simulink model "FOC_LADRC_G474_bias_isolated_v2"  (R2020b)
settings: Solver=FixedStepDiscrete  StartTime=0.0  StopTime=10  FixedStep=TsBSP  RelTol=1e-3
values from neighbouring files (symbols this model uses):
  BandwidthCurrentPI = 1256.6370614359173    [G474_FOC_LADRC.sldd]
  Flux = 0.0109    [G474_FOC_LADRC.sldd]
  Flux_MODEL = 0.0109    [G474_FOC_LADRC.sldd]
  LADRC_b0 = 8000.0    [G474_FOC_LADRC.sldd]
  LADRC_Omega_c = 150.0    [G474_FOC_LADRC.sldd]
  Ls = 0.000195185    [G474_FOC_LADRC.sldd]
  MaxVoltage = 10.0    [G474_FOC_LADRC.sldd]
  pll_omega = 5000.0    [G474_FOC_LADRC.sldd]
  pll_xi = 10.0    [G474_FOC_LADRC.sldd]
  PolePairs = 5.0    [G474_FOC_LADRC.sldd]
  PolePairs_MODEL = 5.0    [G474_FOC_LADRC.sldd]
  PWMHalfPeriod = 4199.0    [G474_FOC_LADRC.sldd]
  Rs = 0.1763    [G474_FOC_LADRC.sldd]
  TsBSP = 2.5E-5    [G474_FOC_LADRC.sldd]
  TsBSP_MODEL = 2.5E-5    [G474_FOC_LADRC.sldd]
  TsFOC = 0.0001    [G474_FOC_LADRC.sldd]
  TsFOC_MODEL = 0.0001    [G474_FOC_LADRC.sldd]
undefined symbols (not defined in the file or in its folder): DiscIntNeverNeededParam, magnitude, sigbuilder_block
libraries: slpidlib x3, mcbplantlib x1, autolibpmsmexterior x1
PreSaveFcn:
  | cd(fileparts(which(bdroot)));
settings Model: DataDictionary=G474_FOC_LADRC.sldd  PacingRate=1000  Creator=beau_  LastModifiedBy=admin
settings DataIOCC: SaveOutput=off  DSMLogging=off  SaveTime=off  ReturnWorkspaceOutputs=off
settings OptimizationCC: DefaultParameterBehavior=Inlined  EnhancedBackFolding=on  PassReuseOutputArgsAs=Individual arguments  ZeroExternalMemoryAtStartup=off  OptimizeBlockOrder=speed  DifferentSizesBufferReuse=on  OptimizationCustomize=off  EfficientTunableParamExpr=on
settings DebuggingCC: SignalRangeChecking=warning  ParameterPrecisionLossMsg=none  ParameterTunabilityLossMsg=error
settings HardwareCC: ProdBitPerPointer=32  ProdBitPerSizeT=32  ProdBitPerPtrDiffT=32  ProdLargestAtomicInteger=Long  ProdLargestAtomicFloat=Double  ProdWordSize=32  ProdHWDeviceType=ARM Compatible->ARM Cortex-M
settings SFSimCC: SimParseCustomCode=off  MATLABDynamicMemAlloc=off
settings RTWCC: Description=Embedded Coder  SystemTargetFile=ert.tlc  GenCodeOnly=on  TemplateMakefile=ert_default_tmf  RTWUseSimCustomCode=on
settings CodeAppCC: ForceParamTrailComments=on  GenerateComments=off  IgnoreCustomStorageClasses=off  OperatorAnnotations=on  SimulinkDataObjDesc=on  SFDataObjDesc=on  InsertBlockDesc=on
settings ERTTargetCC: TargetLangStandard=C99 (ISO)  CodeReplacementLibrary=ARM Cortex-M  GenerateSampleERTMain=on  SupportAbsoluteTime=off  SupportNonFinite=off  SupportComplex=off  InlinedParameterPlacement=NonHierarchical  ERTCustomFileTemplate=example_file_process.tlc  IndentSize=4

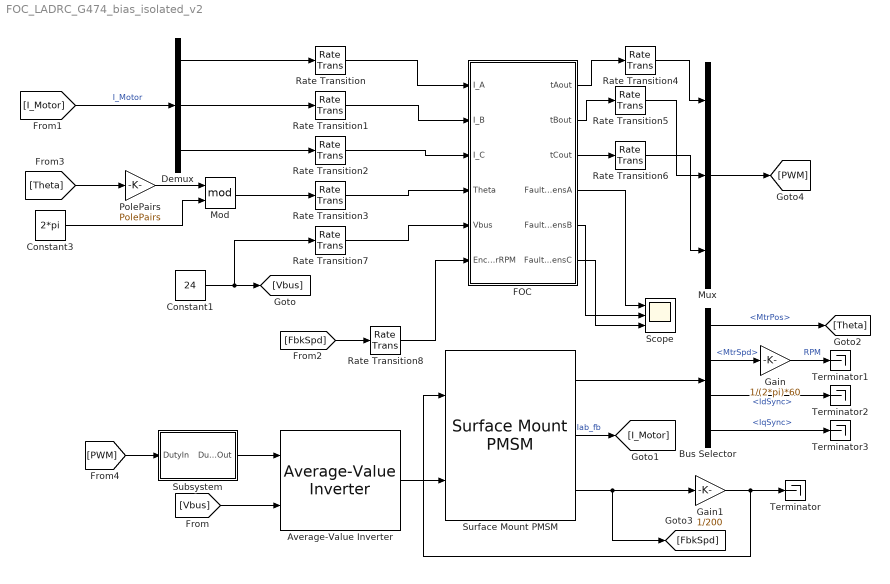
== system FOC_LADRC_G474_bias_isolated_v2 ==
  Average-Value Inverter : mcbplantlib/Average-Value Inverter
  Bus Selector : BusSelector  OutputSignals=MtrPos,MtrSpd,IdSync,IqSync
  Constant1 : Constant  Value=24  SampleTime=TsBSP
  Constant3 : Constant  Value=2*pi  SampleTime=TsBSP
  Demux : Demux  Outputs=3
  FOC : Subsystem  SystemSampleTime=TsFOC
  Gain : Gain  Gain=1/(2*pi)*60
  Gain1 : Gain  Gain=1/200
  Mod : Math  Operator=mod  SaturateOnIntegerOverflow=on
  Mux : Mux  Inputs=3
  PolePairs : Gain  Gain=PolePairs
  Rate Transition{,1..3,7..8} (6 alike) : RateTransition
  Rate Transition4 : RateTransition  OutPortSampleTime=TsBSP
  Rate Transition5 : RateTransition  OutPortSampleTime=TsBSP
  Rate Transition6 : RateTransition  OutPortSampleTime=TsBSP
  Scope : Scope  NumInputPorts=3
  Subsystem : Subsystem
  Surface Mount PMSM : autolibpmsmexterior/Surface Mount PMSM  port_config=Torque  sim_type=Discrete  Ts=TsBSP_MODEL  P=PolePairs_MODEL  Rs=Rs_MODEL  Ldq_=Ls_MODEL  KConstText=Permanent flux linkage constant (lambda_pm):  lambda_pm=Flux_MODEL  Ke=0.0419  Kt=0.061  mechanical=[2.8e-4, 1e-5, 0]  idq0=[0 0]  theta_init=0  omega_init=5  KConst=Flux_MODEL  lambda_pm_calc=Flux_MODEL  RefBlkName='autolibpmsmexterior/Surface Mount PMSM'  aMode=5  Ldq="[0.0017      0.0017]"
      settings: SourceProductBaseCode=PW,MT,UV,VE,VP
  Terminator{,1..3} (4 alike) : Terminator
  wires:
  Average-Value Inverter/1 -> Surface Mount PMSM/2
  Rate Transition4/1 -> Mux/1
  Surface Mount PMSM/2 -> [I_Motor]  "Iab_fb"
  Rate Transition7/1 -> FOC/5(Vbus)
  Surface Mount PMSM/3 -> [FbkSpd], Gain1/1
  Bus Selector/4 -> Terminator3/1  "<IqSync>"
  Bus Selector/3 -> Terminator2/1  "<IdSync>"
  [Vbus] -> Average-Value Inverter/2
  Mux/1 -> [PWM]
  Rate Transition2/1 -> FOC/3(I_C)
  Mod/1 -> Rate Transition3/1
  PolePairs/1 -> Mod/1
  Subsystem/1(DutyOut) -> Average-Value Inverter/1
  Constant1/1 -> Rate Transition7/1, [Vbus]
  Rate Transition3/1 -> FOC/4(Theta)
  Demux/3 -> Rate Transition2/1
  Rate Transition/1 -> FOC/1(I_A)
  Demux/1 -> Rate Transition/1
  Gain1/1 -> Surface Mount PMSM/1, Terminator/1
  Rate Transition5/1 -> Mux/2
  Surface Mount PMSM/1 -> Bus Selector/1
  Rate Transition6/1 -> Mux/3
  Bus Selector/1 -> [Theta]  "<MtrPos>"
  FOC/2(tBout) -> Rate Transition5/1
  [Theta] -> PolePairs/1
  FOC/3(tCout) -> Rate Transition6/1
  FOC/1(tAout) -> Rate Transition4/1
  Demux/2 -> Rate Transition1/1
  Bus Selector/2 -> Gain/1  "<MtrSpd>"
  Constant3/1 -> Mod/2
  Rate Transition1/1 -> FOC/2(I_B)
  [PWM] -> Subsystem/1(DutyIn)
  [I_Motor] -> Demux/1  "I_Motor"
  Gain/1 -> Terminator1/1  "RPM"
  [FbkSpd] -> Rate Transition8/1
  Rate Transition8/1 -> FOC/6(EncoderRPM)
  FOC/4(Fault_ISensA) -> Scope/1
  FOC/5(Fault_ISensB) -> Scope/2
  FOC/6(Fault_ISensC) -> Scope/3

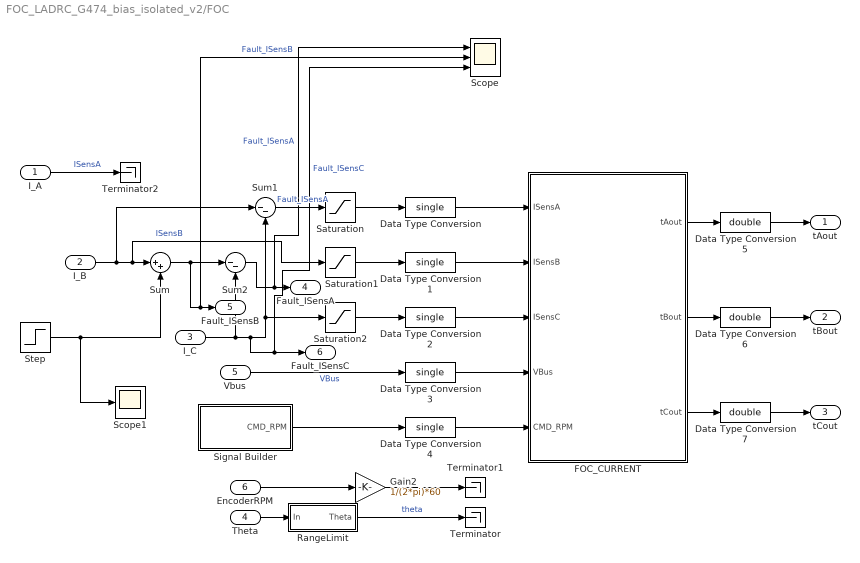
== system FOC_LADRC_G474_bias_isolated_v2/FOC ==
  I_A : Inport
  I_B : Inport  Port=2
  I_C : Inport  Port=3
  Theta : Inport  Port=4
  Vbus : Inport  Port=5
  EncoderRPM : Inport  Port=6
  Data Type Conversion{,1..4} (5 alike) : DataTypeConversion  OutDataTypeStr=single
  Data Type Conversion5 : DataTypeConversion  OutDataTypeStr=double
  Data Type Conversion6 : DataTypeConversion  OutDataTypeStr=double
  Data Type Conversion7 : DataTypeConversion  OutDataTypeStr=double
  FOC_CURRENT : Subsystem  TreatAsAtomicUnit=on  SystemSampleTime=TsFOC_MODEL
  Gain2 : Gain  Gain=1/(2*pi)*60
  RangeLimit : Subsystem
  Saturation : Saturate  UpperLimit=100  LowerLimit=-100
  Saturation1 : Saturate  UpperLimit=100  LowerLimit=-100
  Saturation2 : Saturate  UpperLimit=100  LowerLimit=-100
  Scope : Scope  NumInputPorts=3
  Scope1 : Scope
  Signal Builder : Subsystem  Tag=STV Subsys  LoadFcn=sigbuilder_block('load');  StartFcn=sigbuilder_block('start');  StopFcn=sigbuilder_block('stop');  ClipboardFcn=sigbuilder_block('clipboard');  mask(Sigbuilder block){tuvar=[0:10]}
      mask help: Simulink:masks:SigbuilderBlock_MD
      mask init:
      | if ~strcmp(get_param(bdroot(gcbh),'SimulationStatus'),'stopped') tuvar = sigbuilder_block('maskInit'); end
      settings: CopyFcn=sigbuilder_block('copy');  DeleteFcn=sigbuilder_block('delete');  ModelCloseFcn=sigbuilder_block('modelClose');  PreSaveFcn=sigbuilder_block('preSave');  PauseFcn=sigbuilder_block('pause');  ContinueFcn=sigbuilder_block('continue');  NameChangeFcn=sigbuilder_block('namechange');  OpenFcn=sigbuilder_block('open',[6 65.25 1428 680.25 ]);  CloseFcn=sigbuilder_block('close');
      mask Display: plot(0, 0, 100, 100,[2, 2, 32, 32, 2], [68, 8, 8, 68, 68],[32, 2], [38, 38], [32, 19, 2],[53, 60, 44], [32, 17, 17, 2],[16, 16, 31, 31]);txt = getActiveGroup(gcbh);text(2, 100, txt,'verticalAlignment', 'top');
  Step : Step  Time=3  After=0.5  SampleTime=0
  Sum : Sum  Inputs=|++
  Sum1 : Sum  Inputs=|--
  Sum2 : Sum  Inputs=|--
  Terminator : Terminator
  Terminator1 : Terminator
  Terminator2 : Terminator
  tAout : Outport
  tBout : Outport  Port=2
  tCout : Outport  Port=3
  Fault_ISensA : Outport  Port=4
  Fault_ISensB : Outport  Port=5
  Fault_ISensC : Outport  Port=6
  wires:
  I_C/1 -> Sum2/2, Scope/3, Fault_ISensC/1, Sum1/2, Saturation2/1  "Fault_ISensC"
  Vbus/1 -> Data Type Conversion3/1  "VBus"
  Theta/1 -> RangeLimit/1(In)
  FOC_CURRENT/3(tCout) -> Data Type Conversion7/1
  FOC_CURRENT/1(tAout) -> Data Type Conversion5/1
  FOC_CURRENT/2(tBout) -> Data Type Conversion6/1
  Saturation/1 -> Data Type Conversion/1
  Saturation1/1 -> Data Type Conversion1/1
  Saturation2/1 -> Data Type Conversion2/1
  Signal Builder/1(CMD_RPM) -> Data Type Conversion4/1
  RangeLimit/1(Theta) -> Terminator/1  "theta"
  EncoderRPM/1 -> Gain2/1
  Gain2/1 -> Terminator1/1
  Data Type Conversion/1 -> FOC_CURRENT/1(ISensA)
  Data Type Conversion1/1 -> FOC_CURRENT/2(ISensB)
  Data Type Conversion2/1 -> FOC_CURRENT/3(ISensC)
  Data Type Conversion3/1 -> FOC_CURRENT/4(VBus)
  Data Type Conversion4/1 -> FOC_CURRENT/5(CMD_RPM)
  Data Type Conversion5/1 -> tAout/1
  Data Type Conversion6/1 -> tBout/1
  Data Type Conversion7/1 -> tCout/1
  I_B/1 -> Sum1/1, Saturation1/1, Sum/1  "ISensB"
  Step/1 -> Scope1/1, Sum/2
  Sum1/1 -> Saturation/1  "Fault_ISensA"
  I_A/1 -> Terminator2/1  "ISensA"
  Sum/1 -> Scope/2, Fault_ISensB/1, Sum2/1  "Fault_ISensB"
  Sum2/1 -> Scope/1, Fault_ISensA/1  "Fault_ISensA"

== system FOC_LADRC_G474_bias_isolated_v2/Subsystem ==
  DutyIn : Inport
  Constant : Constant  Value=0.5  SampleTime=TsBSP
  Gain : Gain  Gain=1/PWMHalfPeriod  ParamDataTypeStr=single
  Gain1 : Gain  Gain=-1
  Sum : Sum  Inputs=|+-
  Sum1 : Sum  Inputs=|++
  DutyOut : Outport
  wires:
  Sum/1 -> Gain1/1
  Constant/1 -> Sum1/2, Sum/2
  DutyIn/1 -> Gain/1
  Gain1/1 -> Sum1/1
  Sum1/1 -> DutyOut/1
  Gain/1 -> Sum/1

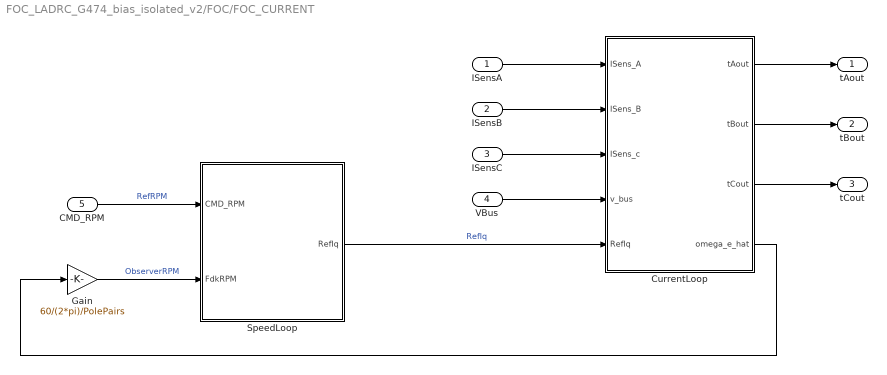
== system FOC_LADRC_G474_bias_isolated_v2/FOC/FOC_CURRENT ==
  ISensA : Inport  OutMin=-100  OutMax=100  OutDataTypeStr=single
  ISensB : Inport  Port=2  OutMin=-100  OutMax=100  OutDataTypeStr=single
  ISensC : Inport  Port=3  OutMin=-100  OutMax=100  OutDataTypeStr=single
  VBus : Inport  Port=4  OutMin=0  OutMax=100  OutDataTypeStr=single
  CMD_RPM : Inport  Port=5  OutDataTypeStr=single
  CurrentLoop : Subsystem
  Gain : Gain  Gain=60/(2*pi)/PolePairs  OutDataTypeStr=single
  SpeedLoop : Subsystem
  tAout : Outport  OutDataTypeStr=single
  tBout : Outport  Port=2  OutDataTypeStr=single
  tCout : Outport  Port=3  OutDataTypeStr=single
  wires:
  SpeedLoop/1(RefIq) -> CurrentLoop/5(RefIq)  "RefIq"
  CMD_RPM/1 -> SpeedLoop/1(CMD_RPM)  "RefRPM"
  Gain/1 -> SpeedLoop/2(FdkRPM)  "ObserverRPM"
  ISensA/1 -> CurrentLoop/1(ISens_A)
  ISensB/1 -> CurrentLoop/2(ISens_B)
  ISensC/1 -> CurrentLoop/3(ISens_c)
  VBus/1 -> CurrentLoop/4(v_bus)
  CurrentLoop/4(omega_e_hat) -> Gain/1
  CurrentLoop/1(tAout) -> tAout/1
  CurrentLoop/2(tBout) -> tBout/1
  CurrentLoop/3(tCout) -> tCout/1

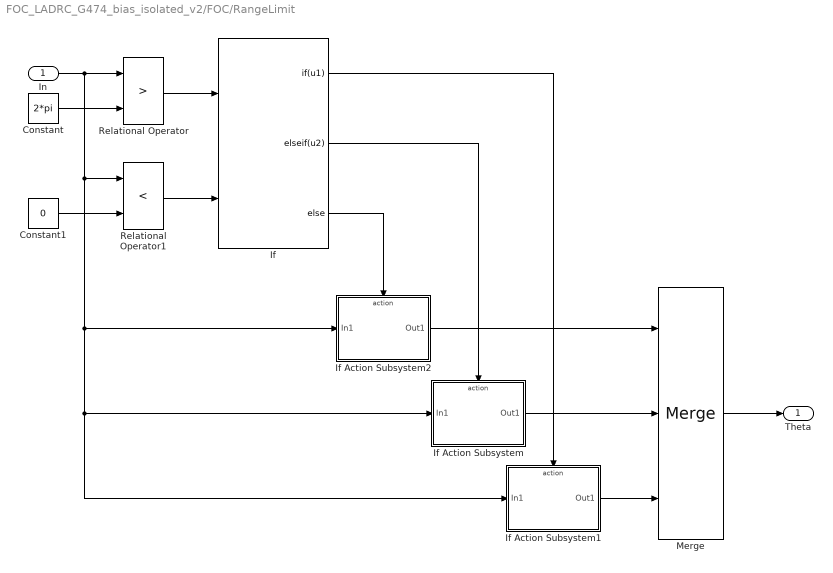
== system FOC_LADRC_G474_bias_isolated_v2/FOC/RangeLimit ==
  In : Inport
  Constant : Constant  Value=2*pi  OutDataTypeStr=single  SampleTime=-1
  Constant1 : Constant  Value=0  OutDataTypeStr=single  SampleTime=-1
  If : If  NumInputs=2  IfExpression=u1  ElseIfExpressions=u2
  If Action Subsystem : Subsystem  TreatAsAtomicUnit=on
  If Action Subsystem1 : Subsystem  TreatAsAtomicUnit=on
  If Action Subsystem2 : Subsystem  TreatAsAtomicUnit=on
  Merge : Merge  Inputs=3
  Relational Operator : RelationalOperator  Operator=>  OutDataTypeStr=boolean  RndMeth=Simplest
  Relational Operator1 : RelationalOperator  Operator=<  OutDataTypeStr=boolean  RndMeth=Simplest
  Theta : Outport
  wires:
  Relational Operator/1 -> If/1
  Constant/1 -> Relational Operator/2
  Constant1/1 -> Relational Operator1/2
  In/1 -> Relational Operator1/1, If Action Subsystem2/1(In1), If Action Subsystem1/1(In1), If Action Subsystem/1(In1), Relational Operator/1
  Relational Operator1/1 -> If/2
  Merge/1 -> Theta/1
  If/3 -> If Action Subsystem2/Action
  If/2 -> If Action Subsystem/Action
  If/1 -> If Action Subsystem1/Action
  If Action Subsystem2/1(Out1) -> Merge/1
  If Action Subsystem/1(Out1) -> Merge/2
  If Action Subsystem1/1(Out1) -> Merge/3

== system FOC_LADRC_G474_bias_isolated_v2/FOC/Signal Builder ==
  Demux : Demux  Tag=STV Demux  Outputs=1
      settings: DisplayOption=none
  FromWs : FromWorkspace  Tag=STV FromWs  VariableName=tuvar
      SigBuilderData=|
      | common.afterFinalStr = 'Extrapolate'
      | common.sampleTime = 0
      | dataSet.timeRange = [0 10]
      | dataSet.name = 'Group 1'
      | sbobj.Groups.Name = 'Group 1'
      | sbobj.Groups.Signals.Name = 'CMD_RPM'
      | sbobj.Groups.Signals.XData = [0 0.52 0.52 1.34 1.34 1.95 1.95 2.4 2.4 3 3 3.41 4 4 5 5 6.01 6.01 7.01 7.01 8 8 9 9 10]
      | sbobj.Groups.Signals.YData = [220 220 1460 1460 500 500 -480 -480 1220 1220 50 50 50 -40 -40 -525 -525 -1015 -1015 50 50 1250 1250 -1325 -1325]
  CMD_RPM : Outport  Tag=STV Outport
  wires:
  FromWs/1 -> Demux/1
  Demux/1 -> CMD_RPM/1

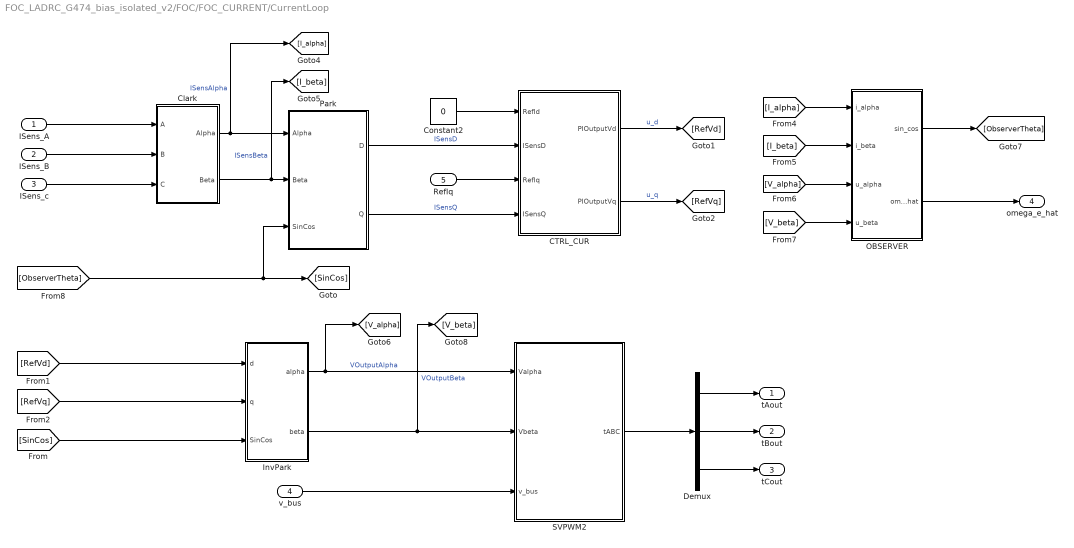
== system FOC_LADRC_G474_bias_isolated_v2/FOC/FOC_CURRENT/CurrentLoop ==
  ISens_A : Inport  OutDataTypeStr=single
  ISens_B : Inport  Port=2  OutDataTypeStr=single
  ISens_c : Inport  Port=3  OutDataTypeStr=single
  v_bus : Inport  Port=4  OutDataTypeStr=single
  RefIq : Inport  Port=5  OutDataTypeStr=single
  CTRL_CUR : Subsystem  TreatAsAtomicUnit=on
  Clark : Subsystem  TreatAsAtomicUnit=on
      settings: RTWSystemCode=Inline  RTWFcnNameOpts=Use subsystem name
      mask Display:
      | port_label('input',1,'a','texmode','on');
      | port_label('input',2,'b','texmode','on');
      | port_label('input',3,'c','texmode','on');
      | 
      | port_label('output',1,'\alpha','texmode','on');
      | port_label('output',2,'\beta','texmode','on');
      | 
      | fprintf('Clark');
  Constant2 : Constant  Value=0  OutDataTypeStr=single
  Demux : Demux  Outputs=3
  InvPark : Subsystem  TreatAsAtomicUnit=on
      settings: RTWFcnNameOpts=Use subsystem name
      mask Display:
      | port_label('input',1,'d','texmode','on');
      | port_label('input',2,'q','texmode','on');
      | port_label('input',3,'\theta','texmode','on');
      | 
      | port_label('output',1,'\alpha','texmode','on');
      | port_label('output',2,'\beta','texmode','on');
      | 
      | fprintf('Inverse\nPark')
  OBSERVER : Subsystem
  Park : Subsystem  TreatAsAtomicUnit=on
      settings: RTWFcnNameOpts=Use subsystem name
      mask Display:
      | port_label('input',1,'\alpha','texmode','on');
      | port_label('input',2, '\beta','texmode','on');
      | port_label('input',3, '\theta','texmode','on');
      | 
      | port_label('output',1,'d','texmode','on');
      | port_label('output',2,'q','texmode','on');
      | fprintf('Park');
  SVPWM2 : Subsystem  TreatAsAtomicUnit=on
  tAout : Outport  OutDataTypeStr=single
  tBout : Outport  Port=2  OutDataTypeStr=single
  tCout : Outport  Port=3  OutDataTypeStr=single
  omega_e_hat : Outport  Port=4  OutDataTypeStr=single
  wires:
  [V_beta] -> OBSERVER/4(u_beta)
  OBSERVER/1(sin_cos) -> [ObserverTheta]
  Clark/2(Beta) -> [I_beta], Park/2(Beta)  "ISensBeta"
  [I_beta] -> OBSERVER/2(i_beta)
  [V_alpha] -> OBSERVER/3(u_alpha)
  Clark/1(Alpha) -> [I_alpha], Park/1(Alpha)  "ISensAlpha"
  ISens_B/1 -> Clark/2(B)
  Demux/3 -> tCout/1
  Constant2/1 -> CTRL_CUR/1(RefId)
  InvPark/1(alpha) -> SVPWM2/1(Valpha), [V_alpha]  "VOutputAlpha"
  [I_alpha] -> OBSERVER/1(i_alpha)
  Park/2(Q) -> CTRL_CUR/4(ISensQ)  "ISensQ"
  [RefVq] -> InvPark/2(q)
  InvPark/2(beta) -> [V_beta], SVPWM2/2(Vbeta)  "VOutputBeta"
  OBSERVER/2(omega_e_hat) -> omega_e_hat/1
  CTRL_CUR/1(PIOutputVd) -> [RefVd]  "u_d"
  v_bus/1 -> SVPWM2/3(v_bus)
  [ObserverTheta] -> Park/3(SinCos), [SinCos]
  Demux/2 -> tBout/1
  Park/1(D) -> CTRL_CUR/2(ISensD)  "ISensD"
  [RefVd] -> InvPark/1(d)
  CTRL_CUR/2(PIOutputVq) -> [RefVq]  "u_q"
  SVPWM2/1(tABC) -> Demux/1
  RefIq/1 -> CTRL_CUR/3(RefIq)
  [SinCos] -> InvPark/3(SinCos)
  Demux/1 -> tAout/1
  ISens_c/1 -> Clark/3(C)
  ISens_A/1 -> Clark/1(A)

== system FOC_LADRC_G474_bias_isolated_v2/FOC/FOC_CURRENT/SpeedLoop ==
  CMD_RPM : Inport  OutDataTypeStr=single
  FdkRPM : Inport  Port=2  OutDataTypeStr=single
  Constant : Constant  Value=LADRC_b0  OutDataTypeStr=single  SampleTime=-1
  Divide : Product  Inputs=*/  OutDataTypeStr=single
  LESO : Subsystem
  Saturation : Saturate  UpperLimit=10  LowerLimit=-10  OutDataTypeStr=single
  Sum : Sum  Inputs=|+-  OutDataTypeStr=single
  Sum1 : Sum  Inputs=|+-  OutDataTypeStr=single
  omega_c : Gain  Gain=LADRC_Omega_c  OutDataTypeStr=single
  RefIq : Outport  OutDataTypeStr=single
  wires:
  Saturation/1 -> RefIq/1, LESO/2(iq)
  Constant/1 -> Divide/2
  Divide/1 -> Saturation/1
  LESO/2(f_hat) -> Sum1/2
  FdkRPM/1 -> LESO/1(FbkSpd)
  LESO/1(omega_r_hat) -> Sum/2
  Sum1/1 -> Divide/1
  omega_c/1 -> Sum1/1
  Sum/1 -> omega_c/1
  CMD_RPM/1 -> Sum/1

== system FOC_LADRC_G474_bias_isolated_v2/FOC/RangeLimit/If Action Subsystem ==
  In1 : Inport
  Action Port : ActionPort  ActionPortLabel=elseif(u2)
  Constant : Constant  Value=2*pi  OutDataTypeStr=single  SampleTime=-1
  Sum : Sum  Inputs=|++
  Out1 : Outport
  wires:
  In1/1 -> Sum/1
  Constant/1 -> Sum/2
  Sum/1 -> Out1/1

== system FOC_LADRC_G474_bias_isolated_v2/FOC/RangeLimit/If Action Subsystem1 ==
  In1 : Inport
  Action Port : ActionPort  ActionPortLabel=if(u1)
  Constant : Constant  Value=2*pi  OutDataTypeStr=single  SampleTime=-1
  Sum : Sum  Inputs=|+-
  Out1 : Outport
  wires:
  In1/1 -> Sum/1
  Constant/1 -> Sum/2
  Sum/1 -> Out1/1

== system FOC_LADRC_G474_bias_isolated_v2/FOC/RangeLimit/If Action Subsystem2 ==
  In1 : Inport
  Action Port : ActionPort  ActionPortLabel=else
  Out1 : Outport
  wires:
  In1/1 -> Out1/1

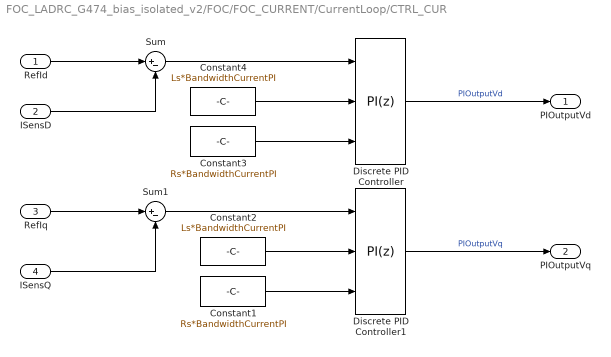
== system FOC_LADRC_G474_bias_isolated_v2/FOC/FOC_CURRENT/CurrentLoop/CTRL_CUR ==
  RefId : Inport  OutDataTypeStr=single
  ISensD : Inport  Port=2  OutDataTypeStr=single
  RefIq : Inport  Port=3  OutDataTypeStr=single
  ISensQ : Inport  Port=4  OutDataTypeStr=single
  Constant1 : Constant  Value=Rs*BandwidthCurrentPI  OutDataTypeStr=single  SampleTime=-1
  Constant2 : Constant  Value=Ls*BandwidthCurrentPI  OutDataTypeStr=single  SampleTime=-1
  Constant3 : Constant  Value=Rs*BandwidthCurrentPI  OutDataTypeStr=single  SampleTime=-1
  Constant4 : Constant  Value=Ls*BandwidthCurrentPI  OutDataTypeStr=single  SampleTime=-1
  Discrete PID Controller : slpidlib/PID Controller  Controller=PI  Form=Parallel  TimeDomain=Discrete-time  UseExternalTs=off  SampleTime=-1  IntegratorMethod=Forward Euler  FilterMethod=Forward Euler  ControllerParametersSource=external  P=1  I=1  D=0  UseFilter=off  N=100  TunerSelectOption=Transfer Function Based (PID Tuner App)  ZeroCross=off  InitialConditionSource=internal  InitialConditionForIntegrator=0  InitialConditionForFilter=0  DifferentiatorICPrevScaledInput=0  ExternalReset=none  TrackingMode=off  Kt=1  LimitOutput=on  SatLimitsSource=internal  UpperSaturationLimit=MaxVoltage  LowerSaturationLimit=-MaxVoltage  LinearizeAsGain=off  AntiWindupMode=clamping  Kb=1  POutMin=[]  POutMax=[]  IOutMin=[]  IOutMax=[]  DOutMin=[]  DOutMax=[]  NOutMin=[]  NOutMax=[]  SumOutMin=[]  SumOutMax=[]  SaturationOutDataTypeStr=Inherit: Inherit via back propagation  SaturationOutMin=[]  SaturationOutMax=[]  PParamMin=[]  PParamMax=[]  IParamMin=[]  IParamMax=[]  DParamMin=[]  DParamMax=[]  NParamMin=[]  NParamMax=[]  KbParamMin=[]  KbParamMax=[]  KtParamMin=[]  KtParamMax=[]  KbOutMin=[]  KbOutMax=[]  KtOutMin=[]  KtOutMax=[]  IntegratorOutMin=[]  IntegratorOutMax=[]  FilterOutMin=[]  FilterOutMax=[]  SumI1OutMin=[]  SumI1OutMax=[]  SumI2OutMin=[]  SumI2OutMax=[]  SumI3OutMin=[]  SumI3OutMax=[]  SumI4OutMin=[]  SumI4OutMax=[]  SumDOutMin=[]  SumDOutMax=[]  DifferentiatorOutMin=[]  DifferentiatorOutMax=[]  FilterDiffOutCoefMin=[]  FilterDiffOutCoefMax=[]  ReciprocalOutMin=[]  ReciprocalOutMax=[]  SumDenOutMin=[]  SumDenOutMax=[]  SumNumOutMin=[]  SumNumOutMax=[]  DivideOutMin=[]  DivideOutMax=[]  UdiffTsProdOutMin=[]  UdiffTsProdOutMax=[]  NTsProdOutMin=[]  NTsProdOutMax=[]  UintegralTsProdOutMin=[]  UintegralTsProdOutMax=[]  UngainTsProdOutMin=[]  UngainTsProdOutMax=[]  IntegratorContinuousStateAttributes=''  IntegratorStateMustResolveToSignalObject=off  IntegratorRTWStateStorageClass=Auto  FilterContinuousStateAttributes=''  FilterStateMustResolveToSignalObject=off  FilterRTWStateStorageClass=Auto  ParallelPVariant=ExternalParameters  IdealPVariant=Disabled  IVariant=ExternalParameters  DVariant=Disabled  IntegratorVariant=Discrete  SatVariant=Enabled  AWVariant=DiscClampingParallel  PCopyVariant=Disabled  TRVariant=Disabled  FdbkBlocksVariant=Forward  IdealPFdbkVariant=Disabled  SatFdbkVariant=Disabled  DerivativeFilterVariant=Disabled  NVariant=Disabled  NCopyVariant=Disabled_SignalSpec  FilterICVariant=Disabled  IntegratorICVariant=InternalICs  ExternalResetVariant=Disabled  TRSumVariant=Passthrough  SumFdbkVariant=Disabled  SumVariant=Sum_PI  TsampFilterVariant=InternalTs  TsampNgainVariant=Passthrough  TsampIntegralVariant=Passthrough  ExternalSaturationOutDataTypeStr=Inherit: Same as second input
  Discrete PID Controller1 : slpidlib/PID Controller  Controller=PI  Form=Parallel  TimeDomain=Discrete-time  UseExternalTs=off  SampleTime=-1  IntegratorMethod=Forward Euler  FilterMethod=Forward Euler  ControllerParametersSource=external  P=1  I=1  D=0  UseFilter=off  N=100  TunerSelectOption=Transfer Function Based (PID Tuner App)  ZeroCross=off  InitialConditionSource=internal  InitialConditionForIntegrator=0  InitialConditionForFilter=0  DifferentiatorICPrevScaledInput=0  ExternalReset=none  TrackingMode=off  Kt=1  LimitOutput=on  SatLimitsSource=internal  UpperSaturationLimit=MaxVoltage  LowerSaturationLimit=-MaxVoltage  LinearizeAsGain=off  AntiWindupMode=clamping  Kb=1  POutMin=[]  POutMax=[]  IOutMin=[]  IOutMax=[]  DOutMin=[]  DOutMax=[]  NOutMin=[]  NOutMax=[]  SumOutMin=[]  SumOutMax=[]  SaturationOutDataTypeStr=Inherit: Inherit via back propagation  SaturationOutMin=[]  SaturationOutMax=[]  PParamMin=[]  PParamMax=[]  IParamMin=[]  IParamMax=[]  DParamMin=[]  DParamMax=[]  NParamMin=[]  NParamMax=[]  KbParamMin=[]  KbParamMax=[]  KtParamMin=[]  KtParamMax=[]  KbOutMin=[]  KbOutMax=[]  KtOutMin=[]  KtOutMax=[]  IntegratorOutMin=[]  IntegratorOutMax=[]  FilterOutMin=[]  FilterOutMax=[]  SumI1OutMin=[]  SumI1OutMax=[]  SumI2OutMin=[]  SumI2OutMax=[]  SumI3OutMin=[]  SumI3OutMax=[]  SumI4OutMin=[]  SumI4OutMax=[]  SumDOutMin=[]  SumDOutMax=[]  DifferentiatorOutMin=[]  DifferentiatorOutMax=[]  FilterDiffOutCoefMin=[]  FilterDiffOutCoefMax=[]  ReciprocalOutMin=[]  ReciprocalOutMax=[]  SumDenOutMin=[]  SumDenOutMax=[]  SumNumOutMin=[]  SumNumOutMax=[]  DivideOutMin=[]  DivideOutMax=[]  UdiffTsProdOutMin=[]  UdiffTsProdOutMax=[]  NTsProdOutMin=[]  NTsProdOutMax=[]  UintegralTsProdOutMin=[]  UintegralTsProdOutMax=[]  UngainTsProdOutMin=[]  UngainTsProdOutMax=[]  IntegratorContinuousStateAttributes=''  IntegratorStateMustResolveToSignalObject=off  IntegratorRTWStateStorageClass=Auto  FilterContinuousStateAttributes=''  FilterStateMustResolveToSignalObject=off  FilterRTWStateStorageClass=Auto  ParallelPVariant=ExternalParameters  IdealPVariant=Disabled  IVariant=ExternalParameters  DVariant=Disabled  IntegratorVariant=Discrete  SatVariant=Enabled  AWVariant=DiscClampingParallel  PCopyVariant=Disabled  TRVariant=Disabled  FdbkBlocksVariant=Forward  IdealPFdbkVariant=Disabled  SatFdbkVariant=Disabled  DerivativeFilterVariant=Disabled  NVariant=Disabled  NCopyVariant=Disabled_SignalSpec  FilterICVariant=Disabled  IntegratorICVariant=InternalICs  ExternalResetVariant=Disabled  TRSumVariant=Passthrough  SumFdbkVariant=Disabled  SumVariant=Sum_PI  TsampFilterVariant=InternalTs  TsampNgainVariant=Passthrough  TsampIntegralVariant=Passthrough  ExternalSaturationOutDataTypeStr=Inherit: Same as second input
  Sum : Sum  Inputs=|+-  OutDataTypeStr=single
  Sum1 : Sum  Inputs=|+-  OutDataTypeStr=single
  PIOutputVd : Outport  OutDataTypeStr=single
  PIOutputVq : Outport  Port=2  OutDataTypeStr=single
  wires:
  RefId/1 -> Sum/1
  Sum/1 -> Discrete PID Controller/1
  Discrete PID Controller/1 -> PIOutputVd/1  "PIOutputVd"
  ISensD/1 -> Sum/2
  Constant4/1 -> Discrete PID Controller/2
  Constant3/1 -> Discrete PID Controller/3
  RefIq/1 -> Sum1/1
  Constant2/1 -> Discrete PID Controller1/2
  Sum1/1 -> Discrete PID Controller1/1
  ISensQ/1 -> Sum1/2
  Constant1/1 -> Discrete PID Controller1/3
  Discrete PID Controller1/1 -> PIOutputVq/1  "PIOutputVq"

== system FOC_LADRC_G474_bias_isolated_v2/FOC/FOC_CURRENT/CurrentLoop/Clark ==
  A : Inport  OutDataTypeStr=single
  B : Inport  Port=2  OutDataTypeStr=single
  C : Inport  Port=3  OutDataTypeStr=single
  Gain : Gain  Gain=2/3  OutDataTypeStr=single
  Gain1 : Gain  Gain=0.5  OutDataTypeStr=single
  Gain2 : Gain  Gain=sqrt(3)/3  OutDataTypeStr=single
  Sum : Sum  Inputs=|++  OutDataTypeStr=single
  Sum1 : Sum  Inputs=|+-  OutDataTypeStr=single
  Sum2 : Sum  Inputs=+-|  OutDataTypeStr=single
  Alpha : Outport  OutDataTypeStr=single
  Beta : Outport  Port=2  OutDataTypeStr=single
  wires:
  Sum/1 -> Gain1/1
  Gain2/1 -> Beta/1
  B/1 -> Sum2/1, Sum/1
  Gain1/1 -> Sum1/2
  Gain/1 -> Alpha/1
  Sum2/1 -> Gain2/1
  C/1 -> Sum2/2, Sum/2
  A/1 -> Sum1/1
  Sum1/1 -> Gain/1

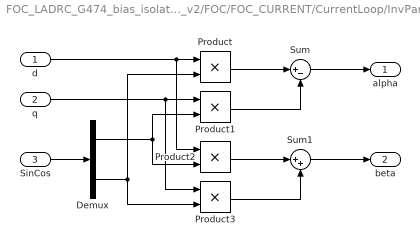
== system FOC_LADRC_G474_bias_isolated_v2/FOC/FOC_CURRENT/CurrentLoop/InvPark ==
  d : Inport  OutDataTypeStr=single
  q : Inport  Port=2  OutDataTypeStr=single
  SinCos : Inport  Port=3  OutDataTypeStr=single
  Demux : Demux  Outputs=2
  Product{,1..3} (4 alike) : Product  OutDataTypeStr=single
  Sum : Sum  Inputs=|+-  OutDataTypeStr=single
  Sum1 : Sum  Inputs=|++  OutDataTypeStr=single
  alpha : Outport  OutDataTypeStr=single
  beta : Outport  Port=2  OutDataTypeStr=single
  wires:
  Sum/1 -> alpha/1
  SinCos/1 -> Demux/1
  d/1 -> Product2/1, Product/1
  Demux/2 -> Product/2, Product3/2
  q/1 -> Product3/1, Product1/1
  Demux/1 -> Product1/2, Product2/2
  Product/1 -> Sum/1
  Product1/1 -> Sum/2
  Product2/1 -> Sum1/1
  Product3/1 -> Sum1/2
  Sum1/1 -> beta/1

== system FOC_LADRC_G474_bias_isolated_v2/FOC/FOC_CURRENT/CurrentLoop/OBSERVER ==
  i_alpha : Inport  OutDataTypeStr=single
  i_beta : Inport  Port=2  OutDataTypeStr=single
  u_alpha : Inport  Port=3  OutDataTypeStr=single
  u_beta : Inport  Port=4  OutDataTypeStr=single
  equ3.12 : Subsystem
  equ3.6 : Subsystem
  equ3.9 : Subsystem
  sin_cos : Outport  OutDataTypeStr=single
  omega_e_hat : Outport  Port=2  OutDataTypeStr=single
  wires:
  i_beta/1 -> equ3.9/4(i_beta), equ3.6/3(i_beta)
  i_alpha/1 -> equ3.6/1(i_alpha), equ3.9/3(i_alpha)
  u_alpha/1 -> equ3.6/2(u_alpha)
  u_beta/1 -> equ3.6/4(u_beta)
  equ3.6/1(y1) -> equ3.9/1(y1)
  equ3.6/2(y2) -> equ3.9/2(y2)
  equ3.9/1(eta_x1_hat) -> equ3.12/1(eta_x1_hat)
  equ3.9/2(eta_x2_hat) -> equ3.12/2(eta_x2_hat)
  equ3.12/1(sin_cos) -> sin_cos/1
  equ3.12/2(omega_e_hat) -> equ3.9/5(omega_e_hat), omega_e_hat/1

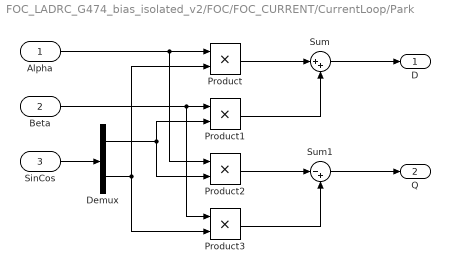
== system FOC_LADRC_G474_bias_isolated_v2/FOC/FOC_CURRENT/CurrentLoop/Park ==
  Alpha : Inport  OutDataTypeStr=single
  Beta : Inport  Port=2  OutDataTypeStr=single
  SinCos : Inport  Port=3  OutDataTypeStr=single
  Demux : Demux  Outputs=2
  Product{,1..3} (4 alike) : Product  OutDataTypeStr=single
  Sum : Sum  Inputs=|++  OutDataTypeStr=single
  Sum1 : Sum  Inputs=|-+  OutDataTypeStr=single
  D : Outport  OutDataTypeStr=single
  Q : Outport  Port=2  OutDataTypeStr=single
  wires:
  Beta/1 -> Product3/1, Product1/1
  Alpha/1 -> Product2/1, Product/1
  SinCos/1 -> Demux/1
  Demux/2 -> Product/2, Product3/2
  Demux/1 -> Product1/2, Product2/2
  Product/1 -> Sum/1
  Product1/1 -> Sum/2
  Sum/1 -> D/1
  Product2/1 -> Sum1/1
  Product3/1 -> Sum1/2
  Sum1/1 -> Q/1

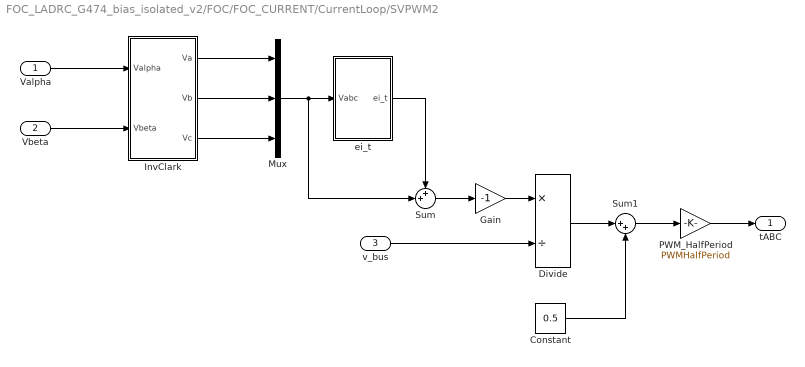
== system FOC_LADRC_G474_bias_isolated_v2/FOC/FOC_CURRENT/CurrentLoop/SVPWM2 ==
  Valpha : Inport  OutDataTypeStr=single
  Vbeta : Inport  Port=2  OutDataTypeStr=single
  v_bus : Inport  Port=3  OutDataTypeStr=single
  Constant : Constant  Value=0.5  OutDataTypeStr=single
  Divide : Product  Inputs=*/  OutDataTypeStr=single
  Gain : Gain  Gain=-1  OutDataTypeStr=single
  InvClark : Subsystem
  Mux : Mux  Inputs=3
  PWM_HalfPeriod : Gain  Gain=PWMHalfPeriod  OutDataTypeStr=single
  Sum : Sum  Inputs=++|  OutDataTypeStr=single
  Sum1 : Sum  Inputs=|++  OutDataTypeStr=single
  ei_t : Subsystem
  tABC : Outport  OutDataTypeStr=single
  wires:
  Valpha/1 -> InvClark/1(Valpha)
  Vbeta/1 -> InvClark/2(Vbeta)
  ei_t/1(ei_t) -> Sum/1
  InvClark/1(Va) -> Mux/1
  InvClark/2(Vb) -> Mux/2
  InvClark/3(Vc) -> Mux/3
  Sum/1 -> Gain/1
  Mux/1 -> Sum/2, ei_t/1(Vabc)
  Divide/1 -> Sum1/1
  Constant/1 -> Sum1/2
  Sum1/1 -> PWM_HalfPeriod/1
  PWM_HalfPeriod/1 -> tABC/1
  v_bus/1 -> Divide/2
  Gain/1 -> Divide/1

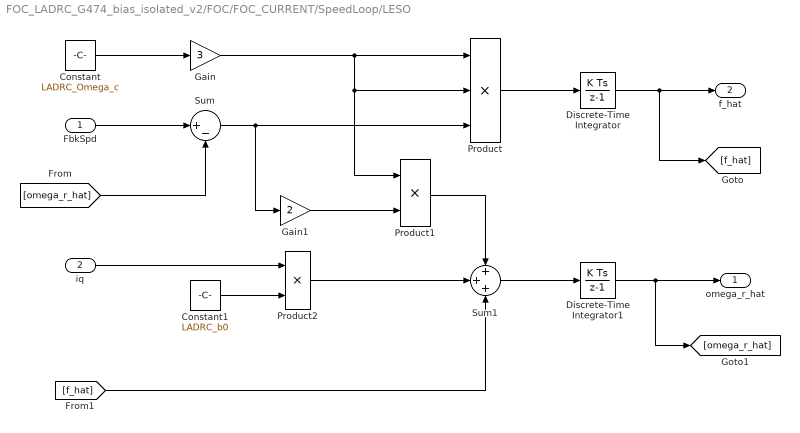
== system FOC_LADRC_G474_bias_isolated_v2/FOC/FOC_CURRENT/SpeedLoop/LESO ==
  FbkSpd : Inport  OutDataTypeStr=single
  iq : Inport  Port=2  OutDataTypeStr=single
  Constant : Constant  Value=LADRC_Omega_c  OutDataTypeStr=single
  Constant1 : Constant  Value=LADRC_b0  OutDataTypeStr=single  SampleTime=-1
  Discrete-Time Integrator : DiscreteIntegrator  SampleTime=-1  OutDataTypeStr=single  UpperSaturationLimit=6e4  LowerSaturationLimit=-6e4  ICPrevOutput=DiscIntNeverNeededParam  ICPrevScaledInput=DiscIntNeverNeededParam
  Discrete-Time Integrator1 : DiscreteIntegrator  SampleTime=-1  OutDataTypeStr=single  LimitOutput=on  UpperSaturationLimit=2000  LowerSaturationLimit=-2000  ICPrevOutput=DiscIntNeverNeededParam  ICPrevScaledInput=DiscIntNeverNeededParam
  Gain : Gain  Gain=3  OutDataTypeStr=single
  Gain1 : Gain  Gain=2  OutDataTypeStr=single
  Product : Product  Inputs=3  OutDataTypeStr=single
  Product1 : Product  OutDataTypeStr=single
  Product2 : Product  OutDataTypeStr=single
  Sum : Sum  Inputs=|+-  OutDataTypeStr=single
  Sum1 : Sum  Inputs=+++  OutDataTypeStr=single
  omega_r_hat : Outport  OutDataTypeStr=single
  f_hat : Outport  Port=2  OutDataTypeStr=single
  wires:
  Sum/1 -> Gain1/1, Product/3
  Product/1 -> Discrete-Time Integrator/1
  Discrete-Time Integrator/1 -> [f_hat], f_hat/1
  [f_hat] -> Sum1/3
  Sum1/1 -> Discrete-Time Integrator1/1
  Discrete-Time Integrator1/1 -> omega_r_hat/1, [omega_r_hat]
  Product1/1 -> Sum1/1
  FbkSpd/1 -> Sum/1
  [omega_r_hat] -> Sum/2
  Constant/1 -> Gain/1
  Gain1/1 -> Product1/2
  Gain/1 -> Product1/1, Product/2, Product/1
  iq/1 -> Product2/1
  Constant1/1 -> Product2/2
  Product2/1 -> Sum1/2

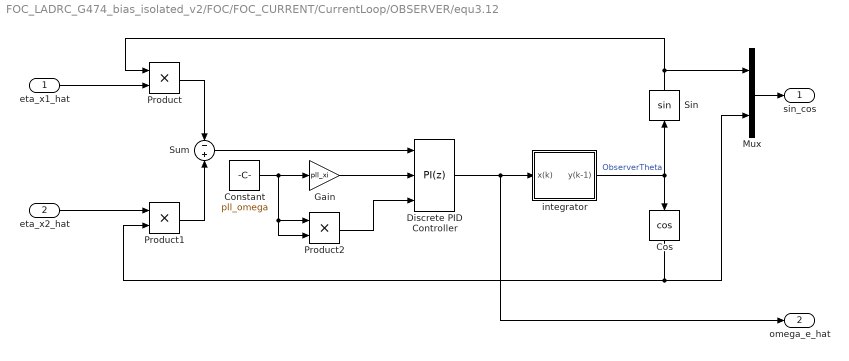
== system FOC_LADRC_G474_bias_isolated_v2/FOC/FOC_CURRENT/CurrentLoop/OBSERVER/equ3.12 ==
  eta_x1_hat : Inport  OutDataTypeStr=single
  eta_x2_hat : Inport  Port=2  OutDataTypeStr=single
  Constant : Constant  Value=pll_omega  OutDataTypeStr=single  SampleTime=-1
  Cos : Trigonometry  Operator=cos
  Discrete PID Controller : slpidlib/PID Controller  Controller=PI  Form=Parallel  TimeDomain=Discrete-time  UseExternalTs=off  SampleTime=-1  IntegratorMethod=Forward Euler  FilterMethod=Forward Euler  ControllerParametersSource=external  P=2*0.707*1650  I=1650*1650  D=0  UseFilter=on  N=100  TunerSelectOption=Transfer Function Based (PID Tuner App)  ZeroCross=off  InitialConditionSource=internal  InitialConditionForIntegrator=0  InitialConditionForFilter=0  DifferentiatorICPrevScaledInput=0  ExternalReset=none  TrackingMode=off  Kt=1  LimitOutput=on  SatLimitsSource=internal  UpperSaturationLimit=2500*2*pi*PolePairs/60  LowerSaturationLimit=-2500*2*pi*PolePairs/60  LinearizeAsGain=off  AntiWindupMode=clamping  Kb=1  POutMin=[]  POutMax=[]  IOutMin=[]  IOutMax=[]  DOutMin=[]  DOutMax=[]  NOutMin=[]  NOutMax=[]  SumOutMin=[]  SumOutMax=[]  SaturationOutMin=[]  SaturationOutMax=[]  PParamMin=[]  PParamMax=[]  IParamMin=[]  IParamMax=[]  DParamMin=[]  DParamMax=[]  NParamMin=[]  NParamMax=[]  KbParamMin=[]  KbParamMax=[]  KtParamMin=[]  KtParamMax=[]  KbOutMin=[]  KbOutMax=[]  KtOutMin=[]  KtOutMax=[]  IntegratorOutMin=[]  IntegratorOutMax=[]  FilterOutMin=[]  FilterOutMax=[]  SumI1OutMin=[]  SumI1OutMax=[]  SumI2OutMin=[]  SumI2OutMax=[]  SumI3OutMin=[]  SumI3OutMax=[]  SumI4OutMin=[]  SumI4OutMax=[]  SumDOutMin=[]  SumDOutMax=[]  DifferentiatorOutMin=[]  DifferentiatorOutMax=[]  FilterDiffOutCoefMin=[]  FilterDiffOutCoefMax=[]  ReciprocalOutMin=[]  ReciprocalOutMax=[]  SumDenOutMin=[]  SumDenOutMax=[]  SumNumOutMin=[]  SumNumOutMax=[]  DivideOutMin=[]  DivideOutMax=[]  UdiffTsProdOutMin=[]  UdiffTsProdOutMax=[]  NTsProdOutMin=[]  NTsProdOutMax=[]  UintegralTsProdOutMin=[]  UintegralTsProdOutMax=[]  UngainTsProdOutMin=[]  UngainTsProdOutMax=[]  IntegratorContinuousStateAttributes=''  IntegratorStateMustResolveToSignalObject=off  IntegratorRTWStateStorageClass=Auto  FilterContinuousStateAttributes=''  FilterStateMustResolveToSignalObject=off  FilterRTWStateStorageClass=Auto  ParallelPVariant=ExternalParameters  IdealPVariant=Disabled  IVariant=ExternalParameters  DVariant=Disabled  IntegratorVariant=Discrete  SatVariant=Enabled  AWVariant=DiscClampingParallel  PCopyVariant=Disabled  TRVariant=Disabled  FdbkBlocksVariant=Forward  IdealPFdbkVariant=Disabled  SatFdbkVariant=Disabled  DerivativeFilterVariant=Disabled  NVariant=Disabled  NCopyVariant=Disabled_SignalSpec  FilterICVariant=Disabled  IntegratorICVariant=InternalICs  ExternalResetVariant=Disabled  TRSumVariant=Passthrough  SumFdbkVariant=Disabled  SumVariant=Sum_PI  TsampFilterVariant=InternalTs  TsampNgainVariant=Passthrough  TsampIntegralVariant=Passthrough  ExternalSaturationOutDataTypeStr=Inherit: Same as second input
  Gain : Gain  Gain=pll_xi  OutDataTypeStr=single
  Mux : Mux  Inputs=2
  Product : Product  OutDataTypeStr=single
  Product1 : Product  OutDataTypeStr=single
  Product2 : Product  OutDataTypeStr=single
  Sin : Trigonometry
  Sum : Sum  Inputs=-|+  OutDataTypeStr=single
  integrator : Subsystem
  sin_cos : Outport  OutDataTypeStr=single
  omega_e_hat : Outport  Port=2  OutDataTypeStr=single
  wires:
  Discrete PID Controller/1 -> omega_e_hat/1, integrator/1(x(k))
  Product/1 -> Sum/1
  Product1/1 -> Sum/2
  Sum/1 -> Discrete PID Controller/1
  Cos/1 -> Product1/2, Mux/2
  Sin/1 -> Mux/1, Product/1
  Mux/1 -> sin_cos/1
  integrator/1(y(k-1)) -> Cos/1, Sin/1  "ObserverTheta"
  eta_x1_hat/1 -> Product/2
  eta_x2_hat/1 -> Product1/1
  Gain/1 -> Discrete PID Controller/2
  Constant/1 -> Product2/2, Product2/1, Gain/1
  Product2/1 -> Discrete PID Controller/3

== system FOC_LADRC_G474_bias_isolated_v2/FOC/FOC_CURRENT/CurrentLoop/OBSERVER/equ3.6 ==
  i_alpha : Inport  OutDataTypeStr=single
  u_alpha : Inport  Port=2  OutDataTypeStr=single
  i_beta : Inport  Port=3  OutDataTypeStr=single
  u_beta : Inport  Port=4  OutDataTypeStr=single
  Add4 : Sum  Inputs=-+  OutDataTypeStr=single
  Add5 : Sum  Inputs=-+  OutDataTypeStr=single
  Gain4 : Gain  Gain=Rs  OutDataTypeStr=single
  Gain5 : Gain  Gain=Rs  OutDataTypeStr=single
  y1 : Outport  OutDataTypeStr=single
  y2 : Outport  Port=2  OutDataTypeStr=single
  wires:
  Add5/1 -> y2/1
  Gain4/1 -> Add4/1
  Gain5/1 -> Add5/1
  u_beta/1 -> Add5/2
  i_beta/1 -> Gain5/1
  Add4/1 -> y1/1
  i_alpha/1 -> Gain4/1
  u_alpha/1 -> Add4/2

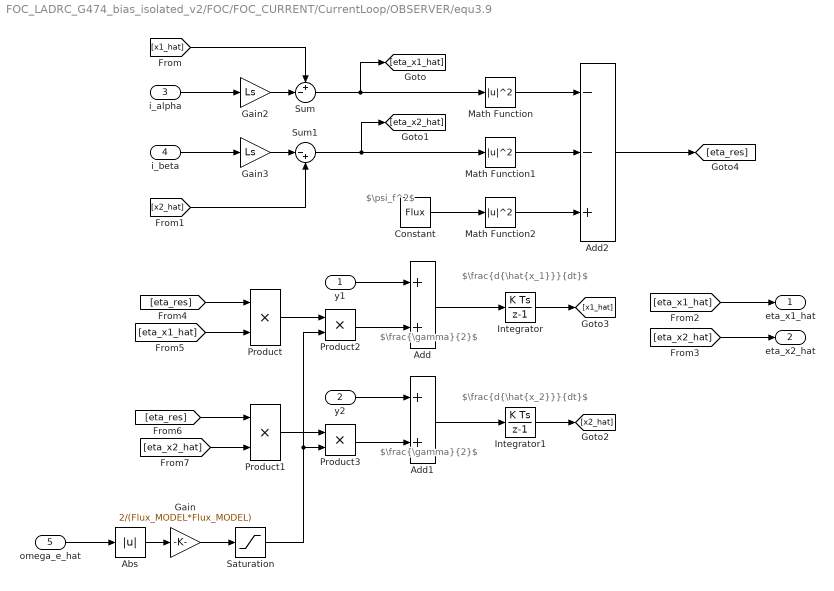
== system FOC_LADRC_G474_bias_isolated_v2/FOC/FOC_CURRENT/CurrentLoop/OBSERVER/equ3.9 ==
  note: $\frac{d{\hat{x_1}}}{dt}$
  note: $\frac{d{\hat{x_2}}}{dt}$
  note: $\frac{\gamma}{2}$
  note: $\frac{\gamma}{2}$
  note: $\psi_f^2$
  y1 : Inport  OutDataTypeStr=single
  y2 : Inport  Port=2  OutDataTypeStr=single
  i_alpha : Inport  Port=3  OutDataTypeStr=single
  i_beta : Inport  Port=4  OutDataTypeStr=single
  omega_e_hat : Inport  Port=5
  Abs : Abs
  Add : Sum  OutDataTypeStr=single
  Add1 : Sum  OutDataTypeStr=single
  Add2 : Sum  Inputs=--+  OutDataTypeStr=single
  Constant : Constant  Value=Flux  OutDataTypeStr=single
  Gain : Gain  Gain=2/(Flux_MODEL*Flux_MODEL)
  Gain2 : Gain  Gain=Ls  OutDataTypeStr=single
  Gain3 : Gain  Gain=Ls  OutDataTypeStr=single
  Integrator : DiscreteIntegrator  SampleTime=-1  OutDataTypeStr=single  ICPrevOutput=DiscIntNeverNeededParam  ICPrevScaledInput=DiscIntNeverNeededParam  mask(DiscretizedDiscreteIntegrator){}
      mask init:
      | %zoh
  Integrator1 : DiscreteIntegrator  SampleTime=-1  OutDataTypeStr=single  ICPrevOutput=DiscIntNeverNeededParam  ICPrevScaledInput=DiscIntNeverNeededParam  mask(DiscretizedDiscreteIntegrator){}
      mask init:
      | %zoh
  Math Function : Math  Operator=magnitude^2  OutDataTypeStr=single  SaturateOnIntegerOverflow=on
  Math Function1 : Math  Operator=magnitude^2  OutDataTypeStr=single  SaturateOnIntegerOverflow=on
  Math Function2 : Math  Operator=magnitude^2  OutDataTypeStr=single  SaturateOnIntegerOverflow=on
  Product : Product  OutDataTypeStr=single
  Product1 : Product  OutDataTypeStr=single
  Product2 : Product
  Product3 : Product
  Saturation : Saturate  UpperLimit=500e4  LowerLimit=10e4
  Sum : Sum  Inputs=+-|  OutDataTypeStr=single
  Sum1 : Sum  Inputs=|-+  OutDataTypeStr=single
  eta_x1_hat : Outport  OutDataTypeStr=single
  eta_x2_hat : Outport  Port=2  OutDataTypeStr=single
  wires:
  y1/1 -> Add/1
  Product3/1 -> Add1/2
  Product1/1 -> Product3/1
  Sum/1 -> [eta_x1_hat], Math Function/1
  Product/1 -> Product2/1
  Product2/1 -> Add/2
  Add/1 -> Integrator/1
  Add1/1 -> Integrator1/1
  Sum1/1 -> Math Function1/1, [eta_x2_hat]
  Integrator1/1 -> [x2_hat]
  y2/1 -> Add1/1
  Integrator/1 -> [x1_hat]
  i_beta/1 -> Gain3/1
  i_alpha/1 -> Gain2/1
  [x2_hat] -> Sum1/2
  Gain3/1 -> Sum1/1
  Math Function1/1 -> Add2/2
  Gain2/1 -> Sum/2
  [x1_hat] -> Sum/1
  Math Function/1 -> Add2/1
  Add2/1 -> [eta_res]
  [eta_x1_hat] -> eta_x1_hat/1
  [eta_x2_hat] -> eta_x2_hat/1
  [eta_res] -> Product/1
  [eta_x1_hat] -> Product/2
  [eta_res] -> Product1/1
  [eta_x2_hat] -> Product1/2
  Constant/1 -> Math Function2/1
  Math Function2/1 -> Add2/3
  omega_e_hat/1 -> Abs/1
  Abs/1 -> Gain/1
  Gain/1 -> Saturation/1
  Saturation/1 -> Product3/2, Product2/2

== system FOC_LADRC_G474_bias_isolated_v2/FOC/FOC_CURRENT/CurrentLoop/SVPWM2/InvClark ==
  Valpha : Inport  OutDataTypeStr=single
  Vbeta : Inport  Port=2  OutDataTypeStr=single
  Gain : Gain  Gain=-1/2  OutDataTypeStr=single
  Gain1 : Gain  Gain=sqrt(3)/2  OutDataTypeStr=single
  Sum : Sum  Inputs=|++  OutDataTypeStr=single
  Sum1 : Sum  Inputs=-+|  OutDataTypeStr=single
  Va : Outport  OutDataTypeStr=single
  Vb : Outport  Port=2  OutDataTypeStr=single
  Vc : Outport  Port=3  OutDataTypeStr=single
  wires:
  Valpha/1 -> Gain/1, Va/1
  Vbeta/1 -> Gain1/1
  Gain/1 -> Sum1/2, Sum/1
  Sum/1 -> Vb/1
  Gain1/1 -> Sum/2, Sum1/1
  Sum1/1 -> Vc/1

== system FOC_LADRC_G474_bias_isolated_v2/FOC/FOC_CURRENT/CurrentLoop/SVPWM2/ei_t ==
  Vabc : Inport  OutDataTypeStr=single
  Demux : Demux  Outputs=3
  Gain : Gain  Gain=-1/2  OutDataTypeStr=single
  Min : MinMax  Inputs=3  OutDataTypeStr=single
  Min1 : MinMax  Function=max  Inputs=3  OutDataTypeStr=single
  Sum : Sum  Inputs=|++  OutDataTypeStr=single
  ei_t : Outport  OutDataTypeStr=single
  wires:
  Min/1 -> Sum/1
  Sum/1 -> Gain/1
  Min1/1 -> Sum/2
  Gain/1 -> ei_t/1
  Vabc/1 -> Demux/1
  Demux/1 -> Min1/1, Min/1
  Demux/2 -> Min/2, Min1/2
  Demux/3 -> Min1/3, Min/3

== system FOC_LADRC_G474_bias_isolated_v2/FOC/FOC_CURRENT/CurrentLoop/OBSERVER/equ3.12/integrator ==
  x(k) : Inport  OutDataTypeStr=single
  RangeLimit : Subsystem
  Sum1 : Sum  Inputs=|++  OutDataTypeStr=single
  Ts : Gain  Gain=TsFOC  OutDataTypeStr=single
  Unit Delay : UnitDelay  SampleTime=-1  HasFrameUpgradeWarning=on
  y(k-1) : Outport  OutDataTypeStr=single
  wires:
  x(k)/1 -> Ts/1
  Ts/1 -> Sum1/1
  Sum1/1 -> RangeLimit/1(In)  "y(k)"
  Unit Delay/1 -> y(k-1)/1, Sum1/2
  RangeLimit/1(Theta) -> Unit Delay/1

== system FOC_LADRC_G474_bias_isolated_v2/FOC/FOC_CURRENT/CurrentLoop/OBSERVER/equ3.12/integrator/RangeLimit ==
  In : Inport  OutDataTypeStr=single
  Constant : Constant  Value=2*pi  OutDataTypeStr=single  SampleTime=-1
  Constant1 : Constant  Value=0  OutDataTypeStr=single  SampleTime=-1
  If : If  NumInputs=2  IfExpression=u1  ElseIfExpressions=u2
  If Action Subsystem : Subsystem  TreatAsAtomicUnit=on
  If Action Subsystem1 : Subsystem  TreatAsAtomicUnit=on
  If Action Subsystem2 : Subsystem  TreatAsAtomicUnit=on
  Merge : Merge  Inputs=3
  Relational Operator : RelationalOperator  Operator=>  OutDataTypeStr=boolean  RndMeth=Simplest
  Relational Operator1 : RelationalOperator  Operator=<  OutDataTypeStr=boolean  RndMeth=Simplest
  Theta : Outport  OutDataTypeStr=single
  wires:
  Relational Operator/1 -> If/1
  Constant/1 -> Relational Operator/2
  Constant1/1 -> Relational Operator1/2
  In/1 -> Relational Operator1/1, If Action Subsystem2/1(In1), If Action Subsystem1/1(In1), If Action Subsystem/1(In1), Relational Operator/1
  Relational Operator1/1 -> If/2
  Merge/1 -> Theta/1
  If/3 -> If Action Subsystem2/Action
  If/2 -> If Action Subsystem/Action
  If/1 -> If Action Subsystem1/Action
  If Action Subsystem2/1(Out1) -> Merge/1
  If Action Subsystem/1(Out1) -> Merge/2
  If Action Subsystem1/1(Out1) -> Merge/3

== system FOC_LADRC_G474_bias_isolated_v2/FOC/FOC_CURRENT/CurrentLoop/OBSERVER/equ3.12/integrator/RangeLimit/If Action Subsystem ==
  In1 : Inport  OutDataTypeStr=single
  Action Port : ActionPort  ActionPortLabel=elseif(u2)
  Constant : Constant  Value=2*pi  OutDataTypeStr=single  SampleTime=-1
  Sum : Sum  Inputs=|++  OutDataTypeStr=single
  Out1 : Outport  OutDataTypeStr=single
  wires:
  In1/1 -> Sum/1
  Constant/1 -> Sum/2
  Sum/1 -> Out1/1

== system FOC_LADRC_G474_bias_isolated_v2/FOC/FOC_CURRENT/CurrentLoop/OBSERVER/equ3.12/integrator/RangeLimit/If Action Subsystem1 ==
  In1 : Inport  OutDataTypeStr=single
  Action Port : ActionPort  ActionPortLabel=if(u1)
  Constant : Constant  Value=2*pi  OutDataTypeStr=single  SampleTime=-1
  Sum : Sum  Inputs=|+-  OutDataTypeStr=single
  Out1 : Outport  OutDataTypeStr=single
  wires:
  In1/1 -> Sum/1
  Constant/1 -> Sum/2
  Sum/1 -> Out1/1

== system FOC_LADRC_G474_bias_isolated_v2/FOC/FOC_CURRENT/CurrentLoop/OBSERVER/equ3.12/integrator/RangeLimit/If Action Subsystem2 ==
  In1 : Inport  OutDataTypeStr=single
  Action Port : ActionPort  ActionPortLabel=else
  Out1 : Outport  OutDataTypeStr=single
  wires:
  In1/1 -> Out1/1
